simulink model "PROVA_SIMULINK"  (R2023b)
settings: Solver=FixedStepDiscrete  StartTime=0.0  StopTime=inf  RelTol=1e-3
PreLoadFcn:
  | try, k = fileparts(get_param(bdroot, 'FileName')); if ~isfile(fullfile(k, 'INIZIA_QUI.m')), k = fileparts(k); end; if ~contains(path, fullfile(k, 'componenti')), addpath(genpath(k)); end; catch, end
libraries: blocchi_telefono x3
settings Model: Creator=simonefildi  LastModifiedBy=simonefildi
settings ModelReferenceCC: UpdateModelReferenceTargets=IfOutOfDate
settings SFSimCC: SimGPUStackLimitPerThread=51200
settings RTWCC: GPUStackLimitPerThread=51200  GPUComputeCapability=7.5
settings ConfigComp: CovMetricSettings=de  CovBoundaryAbsTol=1.0e-5

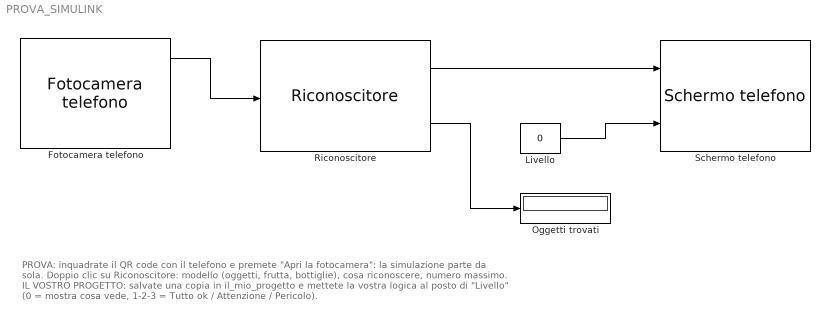
== system PROVA_SIMULINK ==
  note: PROVA: inquadrate il QR code con il telefono e premete "Apri la fotocamera": la simulazione parte da sola.
      | Doppio clic su Riconoscitore: modello (oggetti, frutta, bottiglie), cosa riconoscere, numero massimo.
      | IL VOSTRO PROGETTO: salvate una copia in il_mio_progetto e mettete la vostra logica al posto di "Livello" (0 = mostra cosa vede, 1-2-3 = Tutto ok / Attenzione / Pericolo).
  Fotocamera telefono : blocchi_telefono/Fotocamera telefono  Altezza=640  Larghezza=480  Passo=0.1  AvvioAutomatico=on
      settings: SourceProductName=Telefono e riconoscimento
  Livello : Constant  Value=0
  Oggetti trovati : Display
  Riconoscitore : blocchi_telefono/Riconoscitore  Modello=oggetti  Soglia=0.25  MaxOggetti=10
      settings: SourceProductName=Telefono e riconoscimento
  Schermo telefono : blocchi_telefono/Schermo telefono  Messaggi=Tutto ok|Attenzione|Pericolo  Colori=verde|giallo|rosso
      settings: SourceProductName=Telefono e riconoscimento
  wires:
  Fotocamera telefono/1 -> Riconoscitore/1
  Riconoscitore/1 -> Schermo telefono/1
  Livello/1 -> Schermo telefono/2
  Riconoscitore/2 -> Oggetti trovati/1
